simulink library "WECSim_Lib_Frames"  (R2020b)
settings: Solver=VariableStepAuto  StartTime=0.0  StopTime=10.0  RelTol=1e-3
undefined symbols (not defined in the file or in its folder): simu, waves, X, Y, Z
libraries: sm_lib x8, nesl_utility x2
settings Model: Creator=kmruehl  LastModifiedBy=akeeste

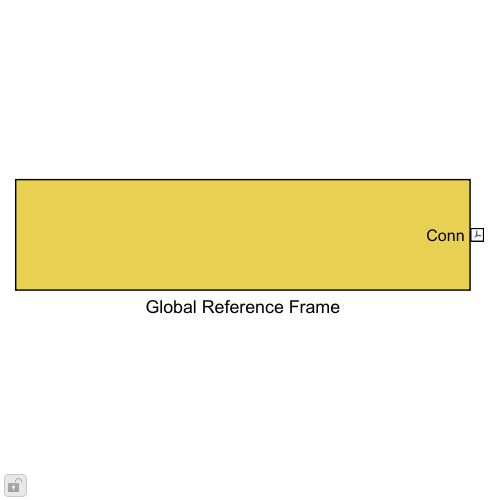
[thumbnail: Simulink's stored preview of the top-level diagram]
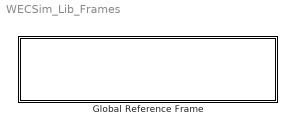
== system WECSim_Lib_Frames ==
  Global Reference Frame : Subsystem  mask(Frames){waves=waves, simu=simu}
      mask prompts: waves "Wave Class Name"; simu "Simulation Class Name"
      mask help:
      | This block contains Global References, including solver configurations, free surface and seabed description, and simulation time.
      | It uses the following fields from the Simulation and Wave classes:
      |
      | Simulation Class:
      |     .endTime
      |     .dt
      |     .domainSize
      |
      | Wave Class:
      |     .waterDepth
      mask Help:
      | This block contains Global References, including solver configurations, free surface and seabed description, and simulation time.
      | It uses the following fields from the Simulation and Wave classes:
      | 
      | Simulation Class:
      |     .endTime
      |     .dt
      |     .domainSize
      | 
      | Wave Class:
      |     .waterDepth

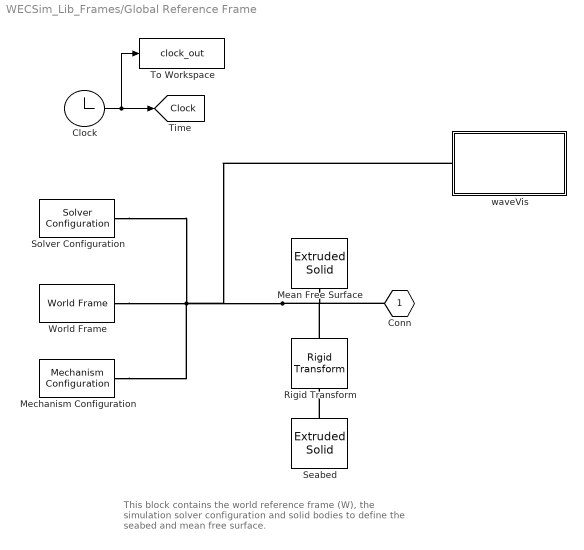
== system WECSim_Lib_Frames/Global Reference Frame ==
  note: This block contains the world reference frame (W), the simulation solver configuration and
      | solid bodies to define the seabed and mean free surface.
  Clock : Clock
  Mean Free Surface : sm_lib/Body Elements/Extruded Solid  ExtrusionType=General  PolygonNumSides=3  PolygonOuterRadius=1  PolygonOuterRadiusUnits=m  ExportEntireGeometry=off  ExtrusionCrossSection=[simu.domainSize simu.domainSize; -simu.domainSize simu.domainSize; -simu.domainSize -simu.domainSize; simu.domainSize -simu.domainSize]  ExtrusionCrossSectionUnits=m  ExportConvexHullGeometry=off  ExtrusionLength=simu.domainSize/200  ExtrusionLengthUnits=m  InertiaType=Custom  BasedOnType=Density  Density=1000  DensityUnits=kg/(m^3)  Mass=10^20  MassUnits=kg  CenterOfMass=[0 0 0]  CenterOfMassUnits=m  MomentsOfInertia=[10^20 10^20 10^20]  MomentsOfInertiaUnits=kg*m^2  ProductsOfInertia=[0 0 0]  ProductsOfInertiaUnits=kg*m^2  GraphicType=FromGeometry  MarkerShape=Sphere  MarkerSize=10  GraphicVisPropType=SimpleVisualProperties  GraphicDiffuseColor=[0.0 0.6 0.8]  GraphicOpacity=0.3  GraphicSpecularColor=[0.5 0.5 0.5 1.0]  GraphicAmbientColor=[0.15 0.15 0.15 1.0]  GraphicEmissiveColor=[0.0 0.0 0.0 1.0]  GraphicShininess=75  DoExposeReferenceFrame=on  SerializedFrames=<Frames/>
  Mechanism Configuration : sm_lib/Utilities/Mechanism Configuration  UniformGravity=Constant  GravityVector=[0 0 0]  GravityVectorUnits=m/s^2  LinearizationDelta=0.001  JointModeTransitionNonlinearIterations=2
  Rigid Transform : sm_lib/Frames and Transforms/Rigid Transform  RotationMethod=None  FollAlignAxisA=+X  BaseAlignAxisA=+Y  FollAlignAxisB=+Y  BaseAlignAxisB=+Z  RotationStandardAxis=+Z  RotationAngle=0  RotationAngleUnits=deg  RotationArbitraryAxis=[0 0 1]  RotationSequenceAxes=FollowerAxes  RotationSequence=XYX  RotationSequenceAngles=[0 0 0]  RotationSequenceAnglesUnits=deg  RotationMatrix=[1 0 0; 0 1 0; 0 0 1]  Quaternion=[1 0 0 0]  TranslationMethod=Cartesian  TranslationCartesianOffset=[0 0 -waves(1).waterDepth]  TranslationCartesianOffsetUnits=m  TranslationStandardAxis=+Z  TranslationStandardOffset=0  TranslationStandardOffsetUnits=m  TranslationROffset=0  TranslationROffsetUnits=m  TranslationThetaOffset=0  TranslationThetaOffsetUnits=deg  TranslationZOffset=0  TranslationZOffsetUnits=m
  Seabed : sm_lib/Body Elements/Extruded Solid  ExtrusionType=General  PolygonNumSides=3  PolygonOuterRadius=1  PolygonOuterRadiusUnits=m  ExportEntireGeometry=off  ExtrusionCrossSection=[simu.domainSize simu.domainSize; -simu.domainSize simu.domainSize; -simu.domainSize -simu.domainSize; simu.domainSize -simu.domainSize]  ExtrusionCrossSectionUnits=m  ExportConvexHullGeometry=off  ExtrusionLength=simu.domainSize/100  ExtrusionLengthUnits=m  InertiaType=Custom  BasedOnType=Density  Density=1000  DensityUnits=kg/(m^3)  Mass=10^20  MassUnits=kg  CenterOfMass=[0 0 0]  CenterOfMassUnits=m  MomentsOfInertia=[10^20 10^20 10^20]  MomentsOfInertiaUnits=kg*m^2  ProductsOfInertia=[0 0 0]  ProductsOfInertiaUnits=kg*m^2  GraphicType=FromGeometry  MarkerShape=Sphere  MarkerSize=10  GraphicVisPropType=SimpleVisualProperties  GraphicDiffuseColor=[0.4 0.4 0.0]  GraphicOpacity=1  GraphicSpecularColor=[0.5 0.5 0.5 1.0]  GraphicAmbientColor=[0.15 0.15 0.15 1.0]  GraphicEmissiveColor=[0.0 0.0 0.0 1.0]  GraphicShininess=75  DoExposeReferenceFrame=on  SerializedFrames=<Frames/>
  Solver Configuration : nesl_utility/Solver Configuration  PhysicalDomain=network_engine_domain  SubClassName=solver  LeftPortType=input  RightPortType=generic  Tones=[]  Harmonics=[]  SimulateNoise=off  Profile=off  UseLocalSampling=off  EnableSwitchedLinearOptims=on  FrequencyDomain=off  UseCCode=off  RelTol=0.001  AbsTol=1e-06  MinStep=1e-09  ToWorkspace=off  RevertToSquareIcSolve=off  NumHomotopyIterations=100  PhasorMode=off  PhasorModeNumHarmonics=1  ConsistencySolver=NEWTON_FTOL  IndexReductionMethod=DerivativeReplacement  DoDC=on  ResidualTolerance=1e-9  ConsistencyTolSource=GLOBAL  ConsistencyAbsTol=0.001  ConsistencyRelTol=0.001  ConsistencyTolFactor=0.001  UseLocalSolver=off  LocalSolverChoice=NE_BACKWARD_EULER_ADVANCER  ResolveIndetEquations=on  FunctionEvalNumThread=1  LocalSolverSampleTime=.001  DoFixedCost=off  MaxNonlinIter=3  MaxModeIter=2  ComputeImpulses=off  ImpulseIterations=2  LinearAlgebra=Sparse  LinearAlgebraNumThread=0  EquationFormulation=NE_TIME_EF  DelaysMemoryBudget=1024  AutomaticFiltering=on  FilteringTimeConstant=0.001  PartitionStorageMethod=AS_NEEDED  PartitionMemoryBudget=1024  PartitionMethod=FAST  MultibodyUseLocalSolver=off  MultibodyLocalSolverChoice=ODE1  MultibodyLocalSolverSampleTime=0.001
  To Workspace : ToWorkspace  VariableName=clock_out  SaveFormat=Structure With Time  SampleTime=-1
  World Frame : sm_lib/Frames and Transforms/World Frame
  waveVis : Subsystem  Variant=on  VariantControl=Choice  AllowZeroVariantControls=on  PropagateVariantConditions=on
  Conn : PMIOPort  Side=Right
  tag scope: Clock=global
  wires:
  Clock/1 -> [Clock], To Workspace/1
  connections:
  Seabed/RConn1 -- Rigid Transform/RConn1
  Solver Configuration/RConn1 -- Rigid Transform/LConn1 -- Mean Free Surface/RConn1 -- Conn/RConn1 -- waveVis/LConn1 -- Mechanism Configuration/RConn1 -- World Frame/RConn1

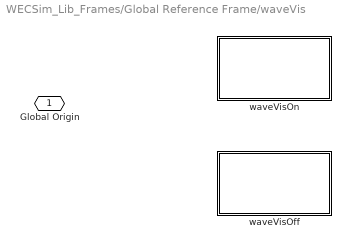
== system WECSim_Lib_Frames/Global Reference Frame/waveVis ==
  waveVisOff : Subsystem  VariantControl=sv_visualizationOFF
  waveVisOn : Subsystem  VariantControl=sv_visualizationON
  Global Origin : PMIOPort  Side=Left

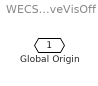
== system WECSim_Lib_Frames/Global Reference Frame/waveVis/waveVisOff ==
  Global Origin : PMIOPort  Side=Left

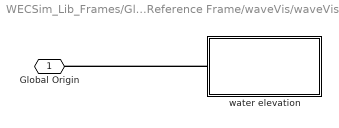
== system WECSim_Lib_Frames/Global Reference Frame/waveVis/waveVisOn ==
  water elevation : Subsystem  mask{waves=waves}
      mask prompts: waves "Waves Object"
      mask init:
      | cb = gcb;
      | nWaves = length(waves);
      | 
      | for i = 1:nWaves
      |     loc = waves(i).marker.location;
      |     nGauges = size(loc,1);
      |     for iWG = 1:nGauges
      |         try 
      |             find_system([cb,'/marker_', num2str(i), num2str(iWG)],'Type','Block');
      |         catch
      |             add_block  ([cb,'/marker1'],[cb,'/marker_', num2str(i), num2str(iWG)],'MakeNameUnique','off',...
      |                        'Position',[0,100*iWG + iWG*3, 180 + iWG*3, 40+100*iWG + iWG*3],'BackgroundColor','white');
      |     
      |             set_param([cb,'/marker_', num2str(i), num2str(iWG)],'wgT',           sprintf('[waves(%d).waveAmpTimeViz(:,1),waves(%d).waveAmpTimeViz(:,%d)]',i,i,iWG+1));
      |     
      |             set_param([cb,'/marker_', num2str(i), num2str(iWG)],'wgloc',         sprintf('waves(%d).marker.location(%d,:)',i,iWG));
      |             
      |             set_param([cb,'/marker_', num2str(i), num2str(iWG)],'markStyle',      sprintf('waves(%d).marker.style',i));
      |     
      |             set_param([cb,'/marker_', num2str(i), num2str(iWG)],'markSize',       sprintf('waves(%d).marker.size',i));
      |     
      |             set_param([cb,'/marker_', num2str(i), num2str(iWG)],'graphicColor',   sprintf('waves(%d).marker.graphicColor',i));
      |     
      |             add_line(cb,...
      |                 ['marker_', num2str(i), num2str(iWG),'/LConn1'],...
      |                 'Global Origin/RConn1',...
      |                 'autorouting','on');
      |         end
      |     end
      | end
  Global Origin : PMIOPort  Side=Left
  connections:
  water elevation/LConn1 -- Global Origin/RConn1

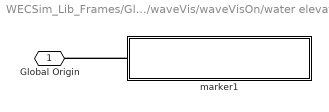
== system WECSim_Lib_Frames/Global Reference Frame/waveVis/waveVisOn/water elevation ==
  marker1 : Subsystem  mask{markStyle=waves(1).marker.style, wgloc=waves(1).marker.location(1,:), wgT=[waves(1).waveAmpTimeViz(:,1), waves(1).waveAmpTimeViz(:,2)], markSize=waves(1).marker.size, graphicColor=waves(1).marker.graphicColor}
      mask prompts: markStyle "Marker Style"; wgloc "Wave Gauge Location [X,Y]"; wgT "Wave Gauge Time History"; markSize "Marker Size"; graphicColor "Graphic Color"
  Global Origin : PMIOPort  Side=Left
  connections:
  marker1/LConn1 -- Global Origin/RConn1

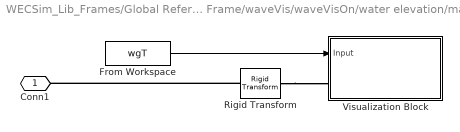
== system WECSim_Lib_Frames/Global Reference Frame/waveVis/waveVisOn/water elevation/marker1 ==
  From Workspace : FromWorkspace  VariableName=wgT
  Rigid Transform : sm_lib/Frames and Transforms/Rigid Transform  RotationMethod=None  FollAlignAxisA=+X  BaseAlignAxisA=+Y  FollAlignAxisB=+Y  BaseAlignAxisB=+Z  RotationStandardAxis=+Z  RotationAngle=0.0  RotationAngleUnits=deg  RotationArbitraryAxis=[0 0 1]  RotationSequenceAxes=FollowerAxes  RotationSequence=XYX  RotationSequenceAngles=[0 0 0]  RotationSequenceAnglesUnits=deg  RotationMatrix=[1 0 0; 0 1 0; 0 0 1]  Quaternion=[1 0 0 0]  TranslationMethod=Cartesian  TranslationCartesianOffset=[wgloc 0]  TranslationCartesianOffsetUnits=m  TranslationStandardAxis=+Z  TranslationStandardOffset=0  TranslationStandardOffsetUnits=m  TranslationROffset=0  TranslationROffsetUnits=m  TranslationThetaOffset=0  TranslationThetaOffsetUnits=deg  TranslationZOffset=0  TranslationZOffsetUnits=m
  Visualization Block : Subsystem  mask{markStyle=markStyle, markSize=markSize, graphicColor=graphicColor}
      mask prompts: markStyle "Waves Marker Style"; markSize "Waves Marker Size"; graphicColor "Graphic Color"
      mask init:
      | % Marker Shape %<MarkerShape>
      | % Marker Size %<MarkerSize>%<MarkerSizeUnits>
      | cb = gcb;
      | 
      | set_param([cb '/WaveElevation'],'MarkerSize','markSize')
      | 
      | if markStyle == 1
      |     set_param([cb '/WaveElevation'],'MarkerShape','Sphere')
      | elseif markStyle == 2
      |     set_param([cb '/WaveElevation'],'MarkerShape','Cube')
      | elseif markStyle == 3
      |     set_param([cb '/WaveElevation'],'MarkerShape','Frame')
      | end
      | set_param([cb '/WaveElevation'],'GraphicDiffuseColor','graphicColor')
      | set_param([cb '/WaveElevation'],'GraphicOpacity','.5')
  Conn1 : PMIOPort  Side=Left
  wires:
  From Workspace/1 -> Visualization Block/1(Input)
  connections:
  Rigid Transform/LConn1 -- Conn1/RConn1
  Rigid Transform/RConn1 -- Visualization Block/LConn1

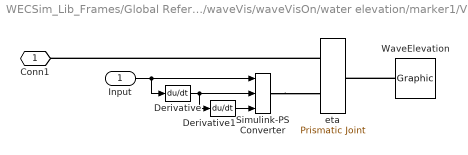
== system WECSim_Lib_Frames/Global Reference Frame/waveVis/waveVisOn/water elevation/marker1/Visualization Block ==
  Input : Inport
  Derivative : Derivative
  Derivative1 : Derivative
  Simulink-PS Converter : nesl_utility/Simulink-PS Converter  PhysicalDomain=network_engine_domain  SubClassName=ps_input  LeftPortType=input  RightPortType=output  PseudoPeriodic=off  Frequencies=[]  NoiseDistribution=none  NoiseParameters=[]  Unit=1  AffineConversion=off  FilteringAndDerivatives=provide  SimscapeFilterOrder=1  InputFilterTimeConstant=0.001  UdotUserProvided=2
  WaveElevation : sm_lib/Body Elements/Graphic  GraphicType=Marker  MarkerShape=Frame  MarkerSize=markSize  GraphicVisPropType=SimpleVisualProperties  GraphicDiffuseColor=graphicColor  GraphicOpacity=.5  GraphicSpecularColor=[0.5 0.5 0.5 1.0]  GraphicAmbientColor=[0.15 0.15 0.15 1.0]  GraphicEmissiveColor=[0.0 0.0 0.0 1.0]  GraphicShininess=75
      settings: AttributesFormatString=|
      | Marker Shape: %<MarkerShape>
      | Marker Size:    %<MarkerSize>%<MarkerSizeUnits>
  eta : sm_lib/Joints/Prismatic Joint  JointMode=Normal  CompositeWrenchDir=FollowerOnBase  CompositeWrenchFrame=BaseFrame  SenseConstraintForce=off  SenseConstraintTorque=off  SenseTotalForce=off  SenseTotalTorque=off  PositionTargetSpecify=off  PositionTargetPriority=High  PositionTargetValue=0  PositionTargetValueUnits=m  VelocityTargetSpecify=off  VelocityTargetPriority=High  VelocityTargetValue=0  VelocityTargetValueUnits=m/s  EquilibriumPosition=0  EquilibriumPositionUnits=m  SpringStiffness=0  SpringStiffnessUnits=N/m  DampingCoefficient=0  DampingCoefficientUnits=N/(m/s)  LowerLimitSpecify=off  LowerLimitBound=-1  LowerLimitBoundUnits=m  LowerLimitStiffness=1e6  LowerLimitStiffnessUnits=N/m  LowerLimitDamping=1e3  LowerLimitDampingUnits=N/(m/s)  LowerLimitTransitionRegionWidth=1e-4  LowerLimitTransitionRegionWidthUnits=m  UpperLimitSpecify=off  UpperLimitBound=1  UpperLimitBoundUnits=m  UpperLimitStiffness=1e6  UpperLimitStiffnessUnits=N/m  UpperLimitDamping=1e3  UpperLimitDampingUnits=N/(m/s)  UpperLimitTransitionRegionWidth=1e-4  UpperLimitTransitionRegionWidthUnits=m  TorqueActuationMode=ComputedTorque  MotionActuationMode=InputMotion  SensePosition=off  SenseVelocity=off  SenseAcceleration=off  SenseTorqueForce=off  SenseLowerLimitTorqueForce=off  SenseUpperLimitTorqueForce=off
  Conn1 : PMIOPort  Side=Left
  wires:
  Derivative1/1 -> Simulink-PS Converter/3
  Derivative/1 -> Simulink-PS Converter/2, Derivative1/1
  Input/1 -> Simulink-PS Converter/1, Derivative/1
  connections:
  eta/LConn1 -- Conn1/RConn1
  WaveElevation/RConn1 -- eta/RConn1
  Simulink-PS Converter/RConn1 -- eta/LConn2
